simulink model "afe_rst_inv_psm_distributed_control_two_delays"  (R2026a)
settings: Solver=ode1be  StopTime=simlength  FixedStep=tc  MaxStep=Tc
values from neighbouring files (symbols this model uses):
  Amplitude_U = 1.16    [grid_fault_generator.m]
  Amplitude_V = Amplitude_U    (= 1.16)    [grid_fault_generator.m]
  Amplitude_W = Amplitude_U    (= 1.16)    [grid_fault_generator.m]
  end_time_LVRT = start_time_LVRT + error_length    [grid_fault_generator.m]
  Igrid_phase_normalization_factor = 270*sqrt(2)    [grid_emulator.m]
  omega_grid_emulator_nom = w_grid    (= 314.159265359)    [grid_emulator.m]
  omega_grid_nom = w_grid    (= 314.159265359)    [grid_emulator.m]
  t_ramp = 20e-3    (= 0.02)    [grid_fault_generator.m]
  ugrid_factor = 1    [grid_emulator.m]
  V_phase_normalization_factor = Vgrid_phase_normalization_factor    [grid_emulator.m]
  Vdc_bez = 1070    [grid_emulator.m]
  Vemu_ref_norm = Vemu_ref * sqrt(2) / V_phase_normalization_factor    [grid_emulator.m]
  vn_eta_pu = 0    [grid_emulator.m]
  vn_xi_pu = 0    [grid_emulator.m]
  vp_xi_pu = 1    [grid_emulator.m]
undefined symbols (not defined in the file or in its folder): Adrso, Aresd, Bresd, CFi, CFu, Cresd, Crso, CTRPIFF_CLIP_RELEASE, dead_time_INV, emf_fb_p, emf_fb_p_ccaller_1, emf_fb_p_ccaller_2, emf_p, emf_p_ccaller_1, emf_p_ccaller_2, fPWM_INV, g0_161Hz, g0_500Hz, g1_161Hz, g1_500Hz, i_grid_neg_eta_lim, i_grid_neg_eta_red_lim, i_grid_neg_xi_lim, i_grid_neg_xi_red_lim, i_grid_pos_eta_lim, i_grid_pos_eta_red_lim, ibez, id_lim, ieta_neg_ref_lim, ieta_pos_ref_lim, iq_lim, ixi_pos_ref_lim, Jm_norm, k_frt_ref, kg, ki_afe, ki_i, ki_id, ki_iq, ki_rc_neg_grid, ki_rc_pos_grid, ki_vs, ki_w, kp_afe, kp_i, kp_id, kp_iq, kp_rc_neg_grid, kp_rc_pos_grid, kp_vs, kp_w, kw, l1, l2, Lalpha_norm, Ld_norm, Ldrso, Lq_norm, Ls_norm, luenberger_l1 ... (+30)
libraries: fl_lib x146, nesl_utility x62, simulink x8, cstblocks_lti x7, sl_discontinuities x3, single_phase_transformer_lib x3, flexshaft_lib x1, permanent_magnet_synchronous_machine x1
(part 3 of 14)

== system afe_rst_inv_psm_distributed_control_two_delays/AFE-Modular/afe_leg_a/solid_state_inverter ==
  Simulink-PS Converter : nesl_utility/Simulink-PS Converter  PhysicalDomain=network_engine_domain  SubClassName=ps_input  LeftPortType=input  RightPortType=output  PseudoPeriodic=off  Frequencies=[]  NoiseDistribution=none  NoiseParameters=[]  Unit=1  AffineConversion=off  FilteringAndDerivatives=provide  SimscapeFilterOrder=1  InputFilterTimeConstant=0.001  UdotUserProvided=0
  Simulink-PS Converter1 : nesl_utility/Simulink-PS Converter  PhysicalDomain=network_engine_domain  SubClassName=ps_input  LeftPortType=input  RightPortType=output  PseudoPeriodic=off  Frequencies=[]  NoiseDistribution=none  NoiseParameters=[]  Unit=1  AffineConversion=off  FilteringAndDerivatives=provide  SimscapeFilterOrder=1  InputFilterTimeConstant=0.001  UdotUserProvided=0
  switch_1 : Subsystem
      settings: PortSchema="{\"entries\":[{\"content\":{\"sides\":[{\"content\":{\"connectorIds\":[\"LConn1\"]},\"type\":\"ConnectorPlacement.EquallySpacedRectSide\",\"uuid\":\"9277da8d-d460-43e6-8478-dd662f15d226\"},{\"content\":{\"connectorIds\":[],\"side\":\"RIGHT\"},\"type\":\"ConnectorPlacement.EquallySpacedRectSide\",\"uuid\":\"a7ece396-f1d9-4f4f-a05b-db1fc65d6e1d\"},{\"content\":{\"connectorIds\":[\"LConn2\"],\"side\":\"TOP\"},\"type\":\"ConnectorPlacement.EquallySpacedRectSide\",\"uuid\":\"fdd70777-e9cf-4317-afb6-cae87f75d5b0\"},{\"content\":{\"connectorIds\":[\"RConn1\"],\"side\":\"BOTTOM\"},\"type\":\"ConnectorPlacement.EquallySpacedRectSide\",\"uuid\":\"2353ed68-b1a1-4775-9ca9-31e268d5443b\"}]},\"type\":\"ConnectorPlacement.EquallySpacedConnector\",\"uuid\":\"d5479f4c-4e65-4791-adcb-73df11f88590\"}],\"packageUris\":[\"http://schema.mathworks.com/mf0/Connector/R2020b\"],\"version\":\"1.0\"}"
  switch_2 : Subsystem
      settings: PortSchema="{\"entries\":[{\"content\":{\"sides\":[{\"content\":{\"connectorIds\":[\"LConn1\"]},\"type\":\"ConnectorPlacement.EquallySpacedRectSide\",\"uuid\":\"9277da8d-d460-43e6-8478-dd662f15d226\"},{\"content\":{\"connectorIds\":[],\"side\":\"RIGHT\"},\"type\":\"ConnectorPlacement.EquallySpacedRectSide\",\"uuid\":\"a7ece396-f1d9-4f4f-a05b-db1fc65d6e1d\"},{\"content\":{\"connectorIds\":[\"LConn2\"],\"side\":\"TOP\"},\"type\":\"ConnectorPlacement.EquallySpacedRectSide\",\"uuid\":\"fdd70777-e9cf-4317-afb6-cae87f75d5b0\"},{\"content\":{\"connectorIds\":[\"RConn1\"],\"side\":\"BOTTOM\"},\"type\":\"ConnectorPlacement.EquallySpacedRectSide\",\"uuid\":\"2353ed68-b1a1-4775-9ca9-31e268d5443b\"}]},\"type\":\"ConnectorPlacement.EquallySpacedConnector\",\"uuid\":\"d5479f4c-4e65-4791-adcb-73df11f88590\"}],\"packageUris\":[\"http://schema.mathworks.com/mf0/Connector/R2020b\"],\"version\":\"1.0\"}"
  Udc(+) : PMIOPort  Side=Left
  us_a : PMIOPort  Port=2  Side=Right
  Udc(-) : PMIOPort  Port=3  Side=Left
  wires:
  [afe_mu_bottom] -> Simulink-PS Converter1/1
  [afe_mu_top] -> Simulink-PS Converter/1
  connections:
  Udc(-)/RConn1 -- switch_2/RConn1
  switch_1/RConn1 -- switch_2/LConn2 -- us_a/RConn1
  Simulink-PS Converter/RConn1 -- switch_1/LConn1
  switch_2/LConn1 -- Simulink-PS Converter1/RConn1
  Udc(+)/RConn1 -- switch_1/LConn2

== system afe_rst_inv_psm_distributed_control_two_delays/AFE-Modular/afe_leg_b/dclink_measure ==
  Controlled Voltage Source : fl_lib/Electrical/Electrical Sources/Controlled Voltage Source
  Current Sensor1 : fl_lib/Electrical/Electrical Sensors/Current Sensor
  Electrical Reference : fl_lib/Electrical/Electrical Elements/Electrical Reference
  Gain : Gain  Gain=107.5e3
  Gain1 : Gain  Gain=1/Vdc_bez
  Quantizer : Quantizer  QuantizationInterval=VoltageQuantization
  Resistor : fl_lib/Electrical/Electrical Elements/Resistor  R=107.5 kOhm  i_specify=off  i_priority=None  i=0 A  i_nominal_specify=off  i_nominal_value=1  i_nominal_unit=A  v_specify=off  v_priority=None  v=0 V  v_nominal_specify=off  v_nominal_value=1  v_nominal_unit=V
  Saturation : Saturate  UpperLimit=inf  LowerLimit=1
  im_udc : nesl_utility/PS-Simulink Converter  PhysicalDomain=network_engine_domain  SubClassName=ps_output  LeftPortType=input  RightPortType=output  PseudoPeriodic=off  Frequencies=[]  VectorFormat=1-D array  Unit=A  AffineConversion=on
  udc : PMIOPort  Side=Left
  tag scope: udc_pu_phase_b=global
  wires:
  Gain1/1 -> [udc_pu_phase_b]
  im_udc/1 -> Gain/1
  Saturation/1 -> Quantizer/1
  Quantizer/1 -> Gain1/1
  Gain/1 -> Saturation/1
  connections:
  Controlled Voltage Source/LConn1 -- Resistor/LConn1
  Resistor/RConn1 -- Current Sensor1/LConn1
  Controlled Voltage Source/RConn2 -- Electrical Reference/LConn1 -- Current Sensor1/RConn2
  Current Sensor1/RConn1 -- im_udc/LConn1
  udc/RConn1 -- Controlled Voltage Source/RConn1

== system afe_rst_inv_psm_distributed_control_two_delays/AFE-Modular/afe_leg_b/driver_board_b ==
  current_ctrl : Subsystem
  dq_pll : Subsystem
  igb_dbb_estimator : Subsystem
  voltage-current-acquisition : Subsystem
  us_alphabeta_ctrl : Outport
  wires:
  current_ctrl/1(us_alphabeta_ctrl) -> us_alphabeta_ctrl/1
  [ixi_ref_dba_fb_dbb] -> current_ctrl/1(i_xi_ref)

== system afe_rst_inv_psm_distributed_control_two_delays/AFE-Modular/afe_leg_b/modulator ==
  us_alphabeta_ctrl : Inport
  Bus Selector : BusSelector  OutputSignals=pwm_v_top,pwm_v_bottom
  Constant1 : Constant
  sv_pwm : Subsystem
  tag scope: afe_mv_bottom=global, afe_mv_top=global
  wires:
  sv_pwm/1(firing_gates) -> Bus Selector/1
  Constant1/1 -> sv_pwm/2(enable)
  Bus Selector/1 -> [afe_mv_top]  "<pwm_v_top>"
  us_alphabeta_ctrl/1 -> sv_pwm/1(ab)
  Bus Selector/2 -> [afe_mv_bottom]  "<pwm_v_bottom>"

== system afe_rst_inv_psm_distributed_control_two_delays/AFE-Modular/afe_leg_b/solid_state_inverter ==
  Simulink-PS Converter : nesl_utility/Simulink-PS Converter  PhysicalDomain=network_engine_domain  SubClassName=ps_input  LeftPortType=input  RightPortType=output  PseudoPeriodic=off  Frequencies=[]  NoiseDistribution=none  NoiseParameters=[]  Unit=1  AffineConversion=off  FilteringAndDerivatives=provide  SimscapeFilterOrder=1  InputFilterTimeConstant=0.001  UdotUserProvided=0
  Simulink-PS Converter1 : nesl_utility/Simulink-PS Converter  PhysicalDomain=network_engine_domain  SubClassName=ps_input  LeftPortType=input  RightPortType=output  PseudoPeriodic=off  Frequencies=[]  NoiseDistribution=none  NoiseParameters=[]  Unit=1  AffineConversion=off  FilteringAndDerivatives=provide  SimscapeFilterOrder=1  InputFilterTimeConstant=0.001  UdotUserProvided=0
  switch_1 : Subsystem
      settings: PortSchema="{\"entries\":[{\"content\":{\"sides\":[{\"content\":{\"connectorIds\":[\"LConn1\"]},\"type\":\"ConnectorPlacement.EquallySpacedRectSide\",\"uuid\":\"9277da8d-d460-43e6-8478-dd662f15d226\"},{\"content\":{\"connectorIds\":[],\"side\":\"RIGHT\"},\"type\":\"ConnectorPlacement.EquallySpacedRectSide\",\"uuid\":\"a7ece396-f1d9-4f4f-a05b-db1fc65d6e1d\"},{\"content\":{\"connectorIds\":[\"LConn2\"],\"side\":\"TOP\"},\"type\":\"ConnectorPlacement.EquallySpacedRectSide\",\"uuid\":\"fdd70777-e9cf-4317-afb6-cae87f75d5b0\"},{\"content\":{\"connectorIds\":[\"RConn1\"],\"side\":\"BOTTOM\"},\"type\":\"ConnectorPlacement.EquallySpacedRectSide\",\"uuid\":\"2353ed68-b1a1-4775-9ca9-31e268d5443b\"}]},\"type\":\"ConnectorPlacement.EquallySpacedConnector\",\"uuid\":\"d5479f4c-4e65-4791-adcb-73df11f88590\"}],\"packageUris\":[\"http://schema.mathworks.com/mf0/Connector/R2020b\"],\"version\":\"1.0\"}"
  switch_2 : Subsystem
      settings: PortSchema="{\"entries\":[{\"content\":{\"sides\":[{\"content\":{\"connectorIds\":[\"LConn1\"]},\"type\":\"ConnectorPlacement.EquallySpacedRectSide\",\"uuid\":\"9277da8d-d460-43e6-8478-dd662f15d226\"},{\"content\":{\"connectorIds\":[],\"side\":\"RIGHT\"},\"type\":\"ConnectorPlacement.EquallySpacedRectSide\",\"uuid\":\"a7ece396-f1d9-4f4f-a05b-db1fc65d6e1d\"},{\"content\":{\"connectorIds\":[\"LConn2\"],\"side\":\"TOP\"},\"type\":\"ConnectorPlacement.EquallySpacedRectSide\",\"uuid\":\"fdd70777-e9cf-4317-afb6-cae87f75d5b0\"},{\"content\":{\"connectorIds\":[\"RConn1\"],\"side\":\"BOTTOM\"},\"type\":\"ConnectorPlacement.EquallySpacedRectSide\",\"uuid\":\"2353ed68-b1a1-4775-9ca9-31e268d5443b\"}]},\"type\":\"ConnectorPlacement.EquallySpacedConnector\",\"uuid\":\"d5479f4c-4e65-4791-adcb-73df11f88590\"}],\"packageUris\":[\"http://schema.mathworks.com/mf0/Connector/R2020b\"],\"version\":\"1.0\"}"
  Udc(+) : PMIOPort  Side=Left
  us_b : PMIOPort  Port=2  Side=Right
  Udc(-) : PMIOPort  Port=3  Side=Left
  wires:
  [afe_mv_top] -> Simulink-PS Converter/1
  [afe_mv_bottom] -> Simulink-PS Converter1/1
  connections:
  Udc(+)/RConn1 -- switch_1/LConn2
  switch_2/LConn1 -- Simulink-PS Converter1/RConn1
  Simulink-PS Converter/RConn1 -- switch_1/LConn1
  switch_2/LConn2 -- us_b/RConn1 -- switch_1/RConn1
  Udc(-)/RConn1 -- switch_2/RConn1

== system afe_rst_inv_psm_distributed_control_two_delays/AFE-Modular/afe_leg_c/dclink_measure ==
  Controlled Voltage Source : fl_lib/Electrical/Electrical Sources/Controlled Voltage Source
  Current Sensor1 : fl_lib/Electrical/Electrical Sensors/Current Sensor
  Electrical Reference : fl_lib/Electrical/Electrical Elements/Electrical Reference
  Gain : Gain  Gain=107.5e3
  Gain1 : Gain  Gain=1/Vdc_bez
  Quantizer : Quantizer  QuantizationInterval=VoltageQuantization
  Resistor : fl_lib/Electrical/Electrical Elements/Resistor  R=107.5 kOhm  i_specify=off  i_priority=None  i=0 A  i_nominal_specify=off  i_nominal_value=1  i_nominal_unit=A  v_specify=off  v_priority=None  v=0 V  v_nominal_specify=off  v_nominal_value=1  v_nominal_unit=V
  Saturation : Saturate  UpperLimit=inf  LowerLimit=1
  im_udc : nesl_utility/PS-Simulink Converter  PhysicalDomain=network_engine_domain  SubClassName=ps_output  LeftPortType=input  RightPortType=output  PseudoPeriodic=off  Frequencies=[]  VectorFormat=1-D array  Unit=A  AffineConversion=on
  udc : PMIOPort  Side=Left
  tag scope: vdc_pu=global
  wires:
  Gain/1 -> Saturation/1
  Quantizer/1 -> Gain1/1
  Saturation/1 -> Quantizer/1
  im_udc/1 -> Gain/1
  Gain1/1 -> [vdc_pu]
  connections:
  udc/RConn1 -- Controlled Voltage Source/RConn1
  Current Sensor1/RConn1 -- im_udc/LConn1
  Current Sensor1/RConn2 -- Electrical Reference/LConn1 -- Controlled Voltage Source/RConn2
  Resistor/RConn1 -- Current Sensor1/LConn1
  Controlled Voltage Source/LConn1 -- Resistor/LConn1

== system afe_rst_inv_psm_distributed_control_two_delays/AFE-Modular/afe_leg_c/driver_board_c ==
  current_ctrl : Subsystem
  dq_pll : Subsystem
  igc_dbc_estimator : Subsystem
  voltage-current-acquisition : Subsystem
  us_alphabeta_ctrl : Outport
  wires:
  current_ctrl/1(us_alphabeta_ctrl) -> us_alphabeta_ctrl/1
  [ixi_ref_dba_fb_dbc] -> current_ctrl/1(i_xi_ref)

== system afe_rst_inv_psm_distributed_control_two_delays/AFE-Modular/afe_leg_c/modulator ==
  u_alphabeta_ctrl : Inport
  Bus Selector : BusSelector  OutputSignals=pwm_w_top,pwm_w_bottom
  Constant1 : Constant
  sv_pwm : Subsystem
  tag scope: afe_mw_bottom=global, afe_mw_top=global
  wires:
  Bus Selector/2 -> [afe_mw_bottom]  "<pwm_w_bottom>"
  u_alphabeta_ctrl/1 -> sv_pwm/1(u_alphabeta_ctrl)
  Bus Selector/1 -> [afe_mw_top]  "<pwm_w_top>"
  Constant1/1 -> sv_pwm/2(enable)
  sv_pwm/1(firing_gates) -> Bus Selector/1

== system afe_rst_inv_psm_distributed_control_two_delays/AFE-Modular/afe_leg_c/solid_state_inverter ==
  Simulink-PS Converter : nesl_utility/Simulink-PS Converter  PhysicalDomain=network_engine_domain  SubClassName=ps_input  LeftPortType=input  RightPortType=output  PseudoPeriodic=off  Frequencies=[]  NoiseDistribution=none  NoiseParameters=[]  Unit=1  AffineConversion=off  FilteringAndDerivatives=provide  SimscapeFilterOrder=1  InputFilterTimeConstant=0.001  UdotUserProvided=0
  Simulink-PS Converter1 : nesl_utility/Simulink-PS Converter  PhysicalDomain=network_engine_domain  SubClassName=ps_input  LeftPortType=input  RightPortType=output  PseudoPeriodic=off  Frequencies=[]  NoiseDistribution=none  NoiseParameters=[]  Unit=1  AffineConversion=off  FilteringAndDerivatives=provide  SimscapeFilterOrder=1  InputFilterTimeConstant=0.001  UdotUserProvided=0
  switch_1 : Subsystem
      settings: PortSchema="{\"entries\":[{\"content\":{\"sides\":[{\"content\":{\"connectorIds\":[\"LConn1\"]},\"type\":\"ConnectorPlacement.EquallySpacedRectSide\",\"uuid\":\"9277da8d-d460-43e6-8478-dd662f15d226\"},{\"content\":{\"connectorIds\":[],\"side\":\"RIGHT\"},\"type\":\"ConnectorPlacement.EquallySpacedRectSide\",\"uuid\":\"a7ece396-f1d9-4f4f-a05b-db1fc65d6e1d\"},{\"content\":{\"connectorIds\":[\"LConn2\"],\"side\":\"TOP\"},\"type\":\"ConnectorPlacement.EquallySpacedRectSide\",\"uuid\":\"fdd70777-e9cf-4317-afb6-cae87f75d5b0\"},{\"content\":{\"connectorIds\":[\"RConn1\"],\"side\":\"BOTTOM\"},\"type\":\"ConnectorPlacement.EquallySpacedRectSide\",\"uuid\":\"2353ed68-b1a1-4775-9ca9-31e268d5443b\"}]},\"type\":\"ConnectorPlacement.EquallySpacedConnector\",\"uuid\":\"d5479f4c-4e65-4791-adcb-73df11f88590\"}],\"packageUris\":[\"http://schema.mathworks.com/mf0/Connector/R2020b\"],\"version\":\"1.0\"}"
  switch_2 : Subsystem
      settings: PortSchema="{\"entries\":[{\"content\":{\"sides\":[{\"content\":{\"connectorIds\":[\"LConn1\"]},\"type\":\"ConnectorPlacement.EquallySpacedRectSide\",\"uuid\":\"9277da8d-d460-43e6-8478-dd662f15d226\"},{\"content\":{\"connectorIds\":[],\"side\":\"RIGHT\"},\"type\":\"ConnectorPlacement.EquallySpacedRectSide\",\"uuid\":\"a7ece396-f1d9-4f4f-a05b-db1fc65d6e1d\"},{\"content\":{\"connectorIds\":[\"LConn2\"],\"side\":\"TOP\"},\"type\":\"ConnectorPlacement.EquallySpacedRectSide\",\"uuid\":\"fdd70777-e9cf-4317-afb6-cae87f75d5b0\"},{\"content\":{\"connectorIds\":[\"RConn1\"],\"side\":\"BOTTOM\"},\"type\":\"ConnectorPlacement.EquallySpacedRectSide\",\"uuid\":\"2353ed68-b1a1-4775-9ca9-31e268d5443b\"}]},\"type\":\"ConnectorPlacement.EquallySpacedConnector\",\"uuid\":\"d5479f4c-4e65-4791-adcb-73df11f88590\"}],\"packageUris\":[\"http://schema.mathworks.com/mf0/Connector/R2020b\"],\"version\":\"1.0\"}"
  Udc(+) : PMIOPort  Side=Left
  us_b : PMIOPort  Port=2  Side=Right
  Udc(-) : PMIOPort  Port=3  Side=Left
  wires:
  [afe_mw_bottom] -> Simulink-PS Converter1/1
  [afe_mw_top] -> Simulink-PS Converter/1
  connections:
  Udc(-)/RConn1 -- switch_2/RConn1
  switch_1/RConn1 -- us_b/RConn1 -- switch_2/LConn2
  Simulink-PS Converter/RConn1 -- switch_1/LConn1
  switch_2/LConn1 -- Simulink-PS Converter1/RConn1
  Udc(+)/RConn1 -- switch_1/LConn2

== system afe_rst_inv_psm_distributed_control_two_delays/FRT-VDE4110/FRT-Detection/dvxi_n//dt ==
  x : Inport
  Gain : Gain  Gain=l2
  Gain1 : Gain  Gain=l1
  Gain5 : Gain  Gain=ts_afe
  Sum : Sum  Inputs=-+|
  Sum1 : Sum  Inputs=|++
  Sum2 : Sum  Inputs=|++
  Sum8 : Sum  Inputs=++|
  Unit Delay1 : UnitDelay  SampleTime=ts_afe
  Unit Delay2 : UnitDelay  SampleTime=ts_afe
  xdot_hat : Outport  VectorParamsAs1DForOutWhenUnconnected=off
  wires:
  Unit Delay2/1 -> Gain5/1, Sum1/2, xdot_hat/1
  Sum8/1 -> Unit Delay1/1
  Sum/1 -> Gain/1, Gain1/1
  Unit Delay1/1 -> Sum/1, Sum2/2  "x_hat"
  Sum2/1 -> Sum8/2
  Gain/1 -> Sum1/1
  Sum1/1 -> Unit Delay2/1
  Gain5/1 -> Sum8/1
  x/1 -> Sum/2  "x"
  Gain1/1 -> Sum2/1

== system afe_rst_inv_psm_distributed_control_two_delays/FRT-VDE4110/FRT-Detection/dvxi_p//dt ==
  x : Inport
  Gain : Gain  Gain=l2
  Gain1 : Gain  Gain=l1
  Gain5 : Gain  Gain=ts_afe
  Sum : Sum  Inputs=-+|
  Sum1 : Sum  Inputs=|++
  Sum2 : Sum  Inputs=|++
  Sum8 : Sum  Inputs=++|
  Unit Delay1 : UnitDelay  SampleTime=ts_afe
  Unit Delay2 : UnitDelay  SampleTime=ts_afe
  xdot_hat : Outport  VectorParamsAs1DForOutWhenUnconnected=off
  wires:
  Gain1/1 -> Sum2/1
  x/1 -> Sum/2  "x"
  Gain5/1 -> Sum8/1
  Sum1/1 -> Unit Delay2/1
  Gain/1 -> Sum1/1
  Sum2/1 -> Sum8/2
  Unit Delay1/1 -> Sum2/2, Sum/1  "x_hat"
  Sum/1 -> Gain1/1, Gain/1
  Sum8/1 -> Unit Delay1/1
  Unit Delay2/1 -> xdot_hat/1, Sum1/2, Gain5/1

== system afe_rst_inv_psm_distributed_control_two_delays/FRT-VDE4110/FRT-PosNegReactiveCurrentReferences/avg_flt_500ms ==
  note: Bei fehler: Alter Grid-Wert wird festgehalten!!
  In1 : Inport
  Constant : Constant  Value=2*pi/500e-3
  Constant1 : Constant  Value=ts_afe
  Constant2 : Constant
  Sum : Sum  Inputs=|-+
  avg_flt_1 : MATLAB Function  TreatAsAtomicUnit=on  SystemSampleTime=ts_afe
  Out1 : Outport  VectorParamsAs1DForOutWhenUnconnected=off
  wires:
  avg_flt_1/1(y1) -> Out1/1  "output"
  Constant1/1 -> avg_flt_1/3(Tc)
  Constant/1 -> avg_flt_1/2(w)
  In1/1 -> avg_flt_1/1(x)  "input"
  Constant2/1 -> Sum/2
  [frt_active] -> Sum/1
  Sum/1 -> avg_flt_1/4(enable)

== system afe_rst_inv_psm_distributed_control_two_delays/FRT-VDE4110/FRT-PosNegReactiveCurrentReferences/avg_flt_500ms1 ==
  note: Bei fehler: Alter Grid-Wert wird festgehalten!!
  In1 : Inport
  Constant : Constant  Value=2*pi/500e-3
  Constant1 : Constant  Value=ts_afe
  avg_flt_1 : MATLAB Function  TreatAsAtomicUnit=on  SystemSampleTime=ts_afe
  Out1 : Outport  VectorParamsAs1DForOutWhenUnconnected=off
  wires:
  avg_flt_1/1(y1) -> Out1/1  "output"
  Constant1/1 -> avg_flt_1/3(Tc)
  Constant/1 -> avg_flt_1/2(w)
  In1/1 -> avg_flt_1/1(x)  "input"
  [frt_active] -> avg_flt_1/4(enable)

== system afe_rst_inv_psm_distributed_control_two_delays/FRT-VDE4110/FRT-PosNegReactiveCurrentReferences/avg_flt_500ms2 ==
  note: Bei fehler: Alter Grid-Wert wird festgehalten!!
  In1 : Inport
  Constant : Constant  Value=2*pi/500e-3
  Constant1 : Constant  Value=ts_afe
  Constant2 : Constant
  Sum : Sum  Inputs=|-+
  avg_flt_1 : MATLAB Function  TreatAsAtomicUnit=on  SystemSampleTime=ts_afe
  Out1 : Outport  VectorParamsAs1DForOutWhenUnconnected=off
  wires:
  avg_flt_1/1(y1) -> Out1/1  "output"
  Constant1/1 -> avg_flt_1/3(Tc)
  Constant/1 -> avg_flt_1/2(w)
  In1/1 -> avg_flt_1/1(x)  "input"
  Constant2/1 -> Sum/2
  [frt_active] -> Sum/1
  Sum/1 -> avg_flt_1/4(enable)

== system afe_rst_inv_psm_distributed_control_two_delays/FRT-VDE4110/FRT-PosNegReactiveCurrentReferences/avg_flt_500ms3 ==
  note: Bei fehler: Alter Grid-Wert wird festgehalten!!
  In1 : Inport
  Constant : Constant  Value=2*pi/500e-3
  Constant1 : Constant  Value=ts_afe
  Constant2 : Constant
  Sum : Sum  Inputs=|-+
  avg_flt_1 : MATLAB Function  TreatAsAtomicUnit=on  SystemSampleTime=ts_afe
  Out1 : Outport  VectorParamsAs1DForOutWhenUnconnected=off
  wires:
  avg_flt_1/1(y1) -> Out1/1  "output"
  Constant1/1 -> avg_flt_1/3(Tc)
  Constant/1 -> avg_flt_1/2(w)
  In1/1 -> avg_flt_1/1(x)  "input"
  [frt_active] -> Sum/1
  Constant2/1 -> Sum/2
  Sum/1 -> avg_flt_1/4(enable)

== system afe_rst_inv_psm_distributed_control_two_delays/FRT-VDE4110/FRT-PosNegReactiveCurrentReferences/u_161Hz_flt1 ==
  input : Inport
  Gain3 : Gain  Gain=g1_161Hz
  Gain6 : Gain  Gain=g0_161Hz
  Sum : Sum  Inputs=|++
  Unit Delay1 : UnitDelay  SampleTime=ts_afe
  output : Outport  VectorParamsAs1DForOutWhenUnconnected=off
  wires:
  Gain6/1 -> Sum/1
  input/1 -> Gain6/1
  Unit Delay1/1 -> Gain3/1
  Gain3/1 -> Sum/2
  Sum/1 -> Unit Delay1/1, output/1

== system afe_rst_inv_psm_distributed_control_two_delays/FRT-VDE4110/FRT-PosNegReactiveCurrentReferences/u_161Hz_flt2 ==
  input : Inport
  Gain3 : Gain  Gain=g1_161Hz
  Gain6 : Gain  Gain=g0_161Hz
  Sum : Sum  Inputs=|++
  Unit Delay1 : UnitDelay  SampleTime=ts_afe
  output : Outport  VectorParamsAs1DForOutWhenUnconnected=off
  wires:
  Sum/1 -> output/1, Unit Delay1/1
  Gain3/1 -> Sum/2
  Unit Delay1/1 -> Gain3/1
  input/1 -> Gain6/1
  Gain6/1 -> Sum/1

== system afe_rst_inv_psm_distributed_control_two_delays/FRT-VDE4110/FRT-PosNegReactiveCurrentReferences/u_161Hz_flt3 ==
  input : Inport
  Gain3 : Gain  Gain=g1_161Hz
  Gain6 : Gain  Gain=g0_161Hz
  Sum : Sum  Inputs=|++
  Unit Delay1 : UnitDelay  SampleTime=ts_afe
  output : Outport  VectorParamsAs1DForOutWhenUnconnected=off
  wires:
  Gain6/1 -> Sum/1
  input/1 -> Gain6/1
  Unit Delay1/1 -> Gain3/1
  Gain3/1 -> Sum/2
  Sum/1 -> Unit Delay1/1, output/1

== system afe_rst_inv_psm_distributed_control_two_delays/INV-Modular/inv_leg_u/dclink_measure ==
  Controlled Voltage Source : fl_lib/Electrical/Electrical Sources/Controlled Voltage Source
  Current Sensor1 : fl_lib/Electrical/Electrical Sensors/Current Sensor
  Electrical Reference : fl_lib/Electrical/Electrical Elements/Electrical Reference
  Gain : Gain  Gain=107.5e3
  Gain1 : Gain  Gain=1/Vdc_bez
  Quantizer : Quantizer  QuantizationInterval=VoltageQuantization
  Resistor : fl_lib/Electrical/Electrical Elements/Resistor  R=107.5 kOhm  i_specify=off  i_priority=None  i=0 A  i_nominal_specify=off  i_nominal_value=1  i_nominal_unit=A  v_specify=off  v_priority=None  v=0 V  v_nominal_specify=off  v_nominal_value=1  v_nominal_unit=V
  Saturation : Saturate  UpperLimit=inf  LowerLimit=1
  im_udc : nesl_utility/PS-Simulink Converter  PhysicalDomain=network_engine_domain  SubClassName=ps_output  LeftPortType=input  RightPortType=output  PseudoPeriodic=off  Frequencies=[]  VectorFormat=1-D array  Unit=A  AffineConversion=on
  udc : PMIOPort  Side=Left
  tag scope: udc_dbu=global, udc_pu_dbu=global
  wires:
  Gain/1 -> [udc_dbu], Saturation/1
  Quantizer/1 -> Gain1/1
  Saturation/1 -> Quantizer/1
  im_udc/1 -> Gain/1
  Gain1/1 -> [udc_pu_dbu]
  connections:
  udc/RConn1 -- Controlled Voltage Source/RConn1
  Current Sensor1/RConn1 -- im_udc/LConn1
  Current Sensor1/RConn2 -- Electrical Reference/LConn1 -- Controlled Voltage Source/RConn2
  Resistor/RConn1 -- Current Sensor1/LConn1
  Controlled Voltage Source/LConn1 -- Resistor/LConn1

== system afe_rst_inv_psm_distributed_control_two_delays/INV-Modular/inv_leg_u/driver_board_u ==
  Gain : Gain  Gain=1/omega_bez
  Rate Limiter : RateLimiter  SampleTimeMode=inherited
  Step : Step  Time=0.1  SampleTime=0
  Variant Source : VariantSource  VariantControls={motor_torque_mode == 0, motor_torque_mode == 1}
  double_integrator_observer : Subsystem
  motor_vector_control : Subsystem
  psm_speed_ctrl : Subsystem
  torque_curve : Subsystem
  torque_curve_pu : Scope  NumInputPorts=3
      settings: SampleTime=tc  ActiveDisplayYMinimum=-1.1044  ActiveDisplayYMaximum=0.12271
  voltage-current-acquisition : Subsystem
  us_alphabeta_ctrl : Outport
  tag scope: motor_phase_mb_fb_dbu_luenberger=global, motor_torque_ref_dbu=global
  wires:
  Step/1 -> Rate Limiter/1
  double_integrator_observer/1(omega_pu_hat) -> psm_speed_ctrl/1(motor_omega)
  motor_vector_control/1(us_alphabeta_ctrl) -> us_alphabeta_ctrl/1
  Rate Limiter/1 -> psm_speed_ctrl/2(motor_omega_ref)
  [motor_phase_mb_fb_dbu] -> double_integrator_observer/1(theta)
  double_integrator_observer/2(theta_hat) -> [motor_phase_mb_fb_dbu_luenberger]  "theta_hat"
  [motor_omega_hat_pu_dbu] -> torque_curve_pu/2, torque_curve/1(rotor speed)  "motor_speed_pu_hat"
  Variant Source/1 -> [motor_torque_ref_dbu], motor_vector_control/1(motor_torque_ref)
  psm_speed_ctrl/1(motor_torque_ref) -> Variant Source/1  "motor_torque_pu_ref"
  torque_curve/1(torque_ref) -> Variant Source/2, torque_curve_pu/1  "motor_torque_pu_ref"
  [omega_elec_pmsm] -> Gain/1
  Gain/1 -> torque_curve_pu/3  "motor_speed_pu"

== system afe_rst_inv_psm_distributed_control_two_delays/INV-Modular/inv_leg_u/modulator ==
  us_alphabeta_ctrl : Inport
  Bus Selector : BusSelector  OutputSignals=pwm_u_top,pwm_u_bottom
  Constant1 : Constant
  sv_pwm : Subsystem
  tag scope: inv_mu_bottom=global, inv_mu_top=global
  wires:
  sv_pwm/1(firing_gates) -> Bus Selector/1
  Constant1/1 -> sv_pwm/2(enable)
  Bus Selector/1 -> [inv_mu_top]  "<pwm_u_top>"
  us_alphabeta_ctrl/1 -> sv_pwm/1(ab)
  Bus Selector/2 -> [inv_mu_bottom]  "<pwm_u_bottom>"

== system afe_rst_inv_psm_distributed_control_two_delays/INV-Modular/inv_leg_u/solid_state_inverter ==
  Simulink-PS Converter : nesl_utility/Simulink-PS Converter  PhysicalDomain=network_engine_domain  SubClassName=ps_input  LeftPortType=input  RightPortType=output  PseudoPeriodic=off  Frequencies=[]  NoiseDistribution=none  NoiseParameters=[]  Unit=1  AffineConversion=off  FilteringAndDerivatives=provide  SimscapeFilterOrder=1  InputFilterTimeConstant=0.001  UdotUserProvided=0
  Simulink-PS Converter1 : nesl_utility/Simulink-PS Converter  PhysicalDomain=network_engine_domain  SubClassName=ps_input  LeftPortType=input  RightPortType=output  PseudoPeriodic=off  Frequencies=[]  NoiseDistribution=none  NoiseParameters=[]  Unit=1  AffineConversion=off  FilteringAndDerivatives=provide  SimscapeFilterOrder=1  InputFilterTimeConstant=0.001  UdotUserProvided=0
  switch_1 : Subsystem
      settings: PortSchema="{\"entries\":[{\"content\":{\"sides\":[{\"content\":{\"connectorIds\":[\"LConn1\"]},\"type\":\"ConnectorPlacement.EquallySpacedRectSide\",\"uuid\":\"9277da8d-d460-43e6-8478-dd662f15d226\"},{\"content\":{\"connectorIds\":[],\"side\":\"RIGHT\"},\"type\":\"ConnectorPlacement.EquallySpacedRectSide\",\"uuid\":\"a7ece396-f1d9-4f4f-a05b-db1fc65d6e1d\"},{\"content\":{\"connectorIds\":[\"LConn2\"],\"side\":\"TOP\"},\"type\":\"ConnectorPlacement.EquallySpacedRectSide\",\"uuid\":\"fdd70777-e9cf-4317-afb6-cae87f75d5b0\"},{\"content\":{\"connectorIds\":[\"RConn1\"],\"side\":\"BOTTOM\"},\"type\":\"ConnectorPlacement.EquallySpacedRectSide\",\"uuid\":\"2353ed68-b1a1-4775-9ca9-31e268d5443b\"}]},\"type\":\"ConnectorPlacement.EquallySpacedConnector\",\"uuid\":\"d5479f4c-4e65-4791-adcb-73df11f88590\"}],\"packageUris\":[\"http://schema.mathworks.com/mf0/Connector/R2020b\"],\"version\":\"1.0\"}"
  switch_2 : Subsystem
      settings: PortSchema="{\"entries\":[{\"content\":{\"sides\":[{\"content\":{\"connectorIds\":[\"LConn1\"]},\"type\":\"ConnectorPlacement.EquallySpacedRectSide\",\"uuid\":\"9277da8d-d460-43e6-8478-dd662f15d226\"},{\"content\":{\"connectorIds\":[],\"side\":\"RIGHT\"},\"type\":\"ConnectorPlacement.EquallySpacedRectSide\",\"uuid\":\"a7ece396-f1d9-4f4f-a05b-db1fc65d6e1d\"},{\"content\":{\"connectorIds\":[\"LConn2\"],\"side\":\"TOP\"},\"type\":\"ConnectorPlacement.EquallySpacedRectSide\",\"uuid\":\"fdd70777-e9cf-4317-afb6-cae87f75d5b0\"},{\"content\":{\"connectorIds\":[\"RConn1\"],\"side\":\"BOTTOM\"},\"type\":\"ConnectorPlacement.EquallySpacedRectSide\",\"uuid\":\"2353ed68-b1a1-4775-9ca9-31e268d5443b\"}]},\"type\":\"ConnectorPlacement.EquallySpacedConnector\",\"uuid\":\"d5479f4c-4e65-4791-adcb-73df11f88590\"}],\"packageUris\":[\"http://schema.mathworks.com/mf0/Connector/R2020b\"],\"version\":\"1.0\"}"
  Udc(+) : PMIOPort  Side=Left
  us_u : PMIOPort  Port=2  Side=Right
  Udc(-) : PMIOPort  Port=3  Side=Left
  wires:
  [inv_mu_top] -> Simulink-PS Converter/1
  [inv_mu_bottom] -> Simulink-PS Converter1/1
  connections:
  Udc(+)/RConn1 -- switch_1/LConn2
  switch_2/LConn1 -- Simulink-PS Converter1/RConn1
  Simulink-PS Converter/RConn1 -- switch_1/LConn1
  us_u/RConn1 -- switch_2/LConn2 -- switch_1/RConn1
  Udc(-)/RConn1 -- switch_2/RConn1

== system afe_rst_inv_psm_distributed_control_two_delays/INV-Modular/inv_leg_v/dclink_measure ==
  Controlled Voltage Source : fl_lib/Electrical/Electrical Sources/Controlled Voltage Source
  Current Sensor1 : fl_lib/Electrical/Electrical Sensors/Current Sensor
  Electrical Reference : fl_lib/Electrical/Electrical Elements/Electrical Reference
  Gain : Gain  Gain=107.5e3
  Gain1 : Gain  Gain=1/Vdc_bez
  Quantizer : Quantizer  QuantizationInterval=VoltageQuantization
  Resistor : fl_lib/Electrical/Electrical Elements/Resistor  R=107.5 kOhm  i_specify=off  i_priority=None  i=0 A  i_nominal_specify=off  i_nominal_value=1  i_nominal_unit=A  v_specify=off  v_priority=None  v=0 V  v_nominal_specify=off  v_nominal_value=1  v_nominal_unit=V
  Saturation : Saturate  UpperLimit=inf  LowerLimit=1
  im_udc : nesl_utility/PS-Simulink Converter  PhysicalDomain=network_engine_domain  SubClassName=ps_output  LeftPortType=input  RightPortType=output  PseudoPeriodic=off  Frequencies=[]  VectorFormat=1-D array  Unit=A  AffineConversion=on
  udc : PMIOPort  Side=Left
  tag scope: udc_dbv=global, udc_pu_dbv=global
  wires:
  Gain/1 -> [udc_dbv], Saturation/1
  Quantizer/1 -> Gain1/1
  Saturation/1 -> Quantizer/1
  im_udc/1 -> Gain/1
  Gain1/1 -> [udc_pu_dbv]
  connections:
  udc/RConn1 -- Controlled Voltage Source/RConn1
  Current Sensor1/RConn1 -- im_udc/LConn1
  Current Sensor1/RConn2 -- Electrical Reference/LConn1 -- Controlled Voltage Source/RConn2
  Resistor/RConn1 -- Current Sensor1/LConn1
  Controlled Voltage Source/LConn1 -- Resistor/LConn1

== system afe_rst_inv_psm_distributed_control_two_delays/INV-Modular/inv_leg_v/driver_board_v ==
  double_integrator_observer : Subsystem
  motor_vector_control : Subsystem
  voltage-current-acquisition : Subsystem
  us_alphabeta_ctrl : Outport
  tag scope: motor_phase_mb_fb_dbv_luenberger=global
  wires:
  motor_vector_control/1(us_alphabeta_ctrl) -> us_alphabeta_ctrl/1
  [motor_torque_ref_dbu_fb_dbv] -> motor_vector_control/1(motor_torque_ref)
  [motor_phase_mb_fb_dbv] -> double_integrator_observer/1(theta)
  double_integrator_observer/2(theta_hat) -> [motor_phase_mb_fb_dbv_luenberger]  "theta_hat"

== system afe_rst_inv_psm_distributed_control_two_delays/INV-Modular/inv_leg_v/modulator ==
  us_alphabeta_ctrl : Inport
  Bus Selector : BusSelector  OutputSignals=pwm_v_top,pwm_v_bottom
  Constant1 : Constant
  sv_pwm : Subsystem
  tag scope: inv_mv_bottom=global, inv_mv_top=global
  wires:
  Bus Selector/2 -> [inv_mv_bottom]  "<pwm_v_bottom>"
  us_alphabeta_ctrl/1 -> sv_pwm/1(ab)
  Bus Selector/1 -> [inv_mv_top]  "<pwm_v_top>"
  Constant1/1 -> sv_pwm/2(enable)
  sv_pwm/1(firing_gates) -> Bus Selector/1

== system afe_rst_inv_psm_distributed_control_two_delays/INV-Modular/inv_leg_v/solid_state_inverter ==
  Simulink-PS Converter : nesl_utility/Simulink-PS Converter  PhysicalDomain=network_engine_domain  SubClassName=ps_input  LeftPortType=input  RightPortType=output  PseudoPeriodic=off  Frequencies=[]  NoiseDistribution=none  NoiseParameters=[]  Unit=1  AffineConversion=off  FilteringAndDerivatives=provide  SimscapeFilterOrder=1  InputFilterTimeConstant=0.001  UdotUserProvided=0
  Simulink-PS Converter1 : nesl_utility/Simulink-PS Converter  PhysicalDomain=network_engine_domain  SubClassName=ps_input  LeftPortType=input  RightPortType=output  PseudoPeriodic=off  Frequencies=[]  NoiseDistribution=none  NoiseParameters=[]  Unit=1  AffineConversion=off  FilteringAndDerivatives=provide  SimscapeFilterOrder=1  InputFilterTimeConstant=0.001  UdotUserProvided=0
  switch_1 : Subsystem
      settings: PortSchema="{\"entries\":[{\"content\":{\"sides\":[{\"content\":{\"connectorIds\":[\"LConn1\"]},\"type\":\"ConnectorPlacement.EquallySpacedRectSide\",\"uuid\":\"9277da8d-d460-43e6-8478-dd662f15d226\"},{\"content\":{\"connectorIds\":[],\"side\":\"RIGHT\"},\"type\":\"ConnectorPlacement.EquallySpacedRectSide\",\"uuid\":\"a7ece396-f1d9-4f4f-a05b-db1fc65d6e1d\"},{\"content\":{\"connectorIds\":[\"LConn2\"],\"side\":\"TOP\"},\"type\":\"ConnectorPlacement.EquallySpacedRectSide\",\"uuid\":\"fdd70777-e9cf-4317-afb6-cae87f75d5b0\"},{\"content\":{\"connectorIds\":[\"RConn1\"],\"side\":\"BOTTOM\"},\"type\":\"ConnectorPlacement.EquallySpacedRectSide\",\"uuid\":\"2353ed68-b1a1-4775-9ca9-31e268d5443b\"}]},\"type\":\"ConnectorPlacement.EquallySpacedConnector\",\"uuid\":\"d5479f4c-4e65-4791-adcb-73df11f88590\"}],\"packageUris\":[\"http://schema.mathworks.com/mf0/Connector/R2020b\"],\"version\":\"1.0\"}"
  switch_2 : Subsystem
      settings: PortSchema="{\"entries\":[{\"content\":{\"sides\":[{\"content\":{\"connectorIds\":[\"LConn1\"]},\"type\":\"ConnectorPlacement.EquallySpacedRectSide\",\"uuid\":\"9277da8d-d460-43e6-8478-dd662f15d226\"},{\"content\":{\"connectorIds\":[],\"side\":\"RIGHT\"},\"type\":\"ConnectorPlacement.EquallySpacedRectSide\",\"uuid\":\"a7ece396-f1d9-4f4f-a05b-db1fc65d6e1d\"},{\"content\":{\"connectorIds\":[\"LConn2\"],\"side\":\"TOP\"},\"type\":\"ConnectorPlacement.EquallySpacedRectSide\",\"uuid\":\"fdd70777-e9cf-4317-afb6-cae87f75d5b0\"},{\"content\":{\"connectorIds\":[\"RConn1\"],\"side\":\"BOTTOM\"},\"type\":\"ConnectorPlacement.EquallySpacedRectSide\",\"uuid\":\"2353ed68-b1a1-4775-9ca9-31e268d5443b\"}]},\"type\":\"ConnectorPlacement.EquallySpacedConnector\",\"uuid\":\"d5479f4c-4e65-4791-adcb-73df11f88590\"}],\"packageUris\":[\"http://schema.mathworks.com/mf0/Connector/R2020b\"],\"version\":\"1.0\"}"
  Udc(+) : PMIOPort  Side=Left
  us_u : PMIOPort  Port=2  Side=Right
  Udc(-) : PMIOPort  Port=3  Side=Left
  wires:
  [inv_mv_bottom] -> Simulink-PS Converter1/1
  [inv_mv_top] -> Simulink-PS Converter/1
  connections:
  Udc(-)/RConn1 -- switch_2/RConn1
  switch_1/RConn1 -- switch_2/LConn2 -- us_u/RConn1
  Simulink-PS Converter/RConn1 -- switch_1/LConn1
  switch_2/LConn1 -- Simulink-PS Converter1/RConn1
  Udc(+)/RConn1 -- switch_1/LConn2

== system afe_rst_inv_psm_distributed_control_two_delays/INV-Modular/inv_leg_w/dclink_measure ==
  Controlled Voltage Source : fl_lib/Electrical/Electrical Sources/Controlled Voltage Source
  Current Sensor1 : fl_lib/Electrical/Electrical Sensors/Current Sensor
  Electrical Reference : fl_lib/Electrical/Electrical Elements/Electrical Reference
  Gain : Gain  Gain=107.5e3
  Gain1 : Gain  Gain=1/Vdc_bez
  Quantizer : Quantizer  QuantizationInterval=VoltageQuantization
  Resistor : fl_lib/Electrical/Electrical Elements/Resistor  R=107.5 kOhm  i_specify=off  i_priority=None  i=0 A  i_nominal_specify=off  i_nominal_value=1  i_nominal_unit=A  v_specify=off  v_priority=None  v=0 V  v_nominal_specify=off  v_nominal_value=1  v_nominal_unit=V
  Saturation : Saturate  UpperLimit=inf  LowerLimit=1
  im_udc : nesl_utility/PS-Simulink Converter  PhysicalDomain=network_engine_domain  SubClassName=ps_output  LeftPortType=input  RightPortType=output  PseudoPeriodic=off  Frequencies=[]  VectorFormat=1-D array  Unit=A  AffineConversion=on
  udc : PMIOPort  Side=Left
  tag scope: udc_pu_dbw=global
  wires:
  Gain/1 -> Saturation/1
  Quantizer/1 -> Gain1/1
  Saturation/1 -> Quantizer/1
  im_udc/1 -> Gain/1
  Gain1/1 -> [udc_pu_dbw]
  connections:
  udc/RConn1 -- Controlled Voltage Source/RConn1
  Current Sensor1/RConn1 -- im_udc/LConn1
  Current Sensor1/RConn2 -- Electrical Reference/LConn1 -- Controlled Voltage Source/RConn2
  Resistor/RConn1 -- Current Sensor1/LConn1
  Controlled Voltage Source/LConn1 -- Resistor/LConn1

== system afe_rst_inv_psm_distributed_control_two_delays/INV-Modular/inv_leg_w/driver_board_w ==
  double_integrator_observer : Subsystem
  motor_vector_control : Subsystem
  voltage-current-acquisition : Subsystem
  us_alphabeta_ctrl : Outport
  tag scope: motor_phase_mb_fb_dbw_luenberger=global
  wires:
  [motor_torque_ref_dbu_fb_dbw] -> motor_vector_control/1(motor_torque_ref)
  motor_vector_control/1(us_alphabeta_ctrl) -> us_alphabeta_ctrl/1
  [motor_phase_mb_fb_dbw] -> double_integrator_observer/1(theta)
  double_integrator_observer/2(theta_hat) -> [motor_phase_mb_fb_dbw_luenberger]  "theta_hat"

== system afe_rst_inv_psm_distributed_control_two_delays/INV-Modular/inv_leg_w/modulator ==
  u_alphabeta_ctrl : Inport
  Bus Selector : BusSelector  OutputSignals=pwm_w_top,pwm_w_bottom
  Constant1 : Constant
  sv_pwm : Subsystem
  tag scope: inv_mw_bottom=global, inv_mw_top=global
  wires:
  sv_pwm/1(firing_gates) -> Bus Selector/1
  Constant1/1 -> sv_pwm/2(enable)
  Bus Selector/1 -> [inv_mw_top]  "<pwm_w_top>"
  u_alphabeta_ctrl/1 -> sv_pwm/1(u_alphabeta_ctrl)
  Bus Selector/2 -> [inv_mw_bottom]  "<pwm_w_bottom>"

== system afe_rst_inv_psm_distributed_control_two_delays/INV-Modular/inv_leg_w/solid_state_inverter ==
  Simulink-PS Converter : nesl_utility/Simulink-PS Converter  PhysicalDomain=network_engine_domain  SubClassName=ps_input  LeftPortType=input  RightPortType=output  PseudoPeriodic=off  Frequencies=[]  NoiseDistribution=none  NoiseParameters=[]  Unit=1  AffineConversion=off  FilteringAndDerivatives=provide  SimscapeFilterOrder=1  InputFilterTimeConstant=0.001  UdotUserProvided=0
  Simulink-PS Converter1 : nesl_utility/Simulink-PS Converter  PhysicalDomain=network_engine_domain  SubClassName=ps_input  LeftPortType=input  RightPortType=output  PseudoPeriodic=off  Frequencies=[]  NoiseDistribution=none  NoiseParameters=[]  Unit=1  AffineConversion=off  FilteringAndDerivatives=provide  SimscapeFilterOrder=1  InputFilterTimeConstant=0.001  UdotUserProvided=0
  switch_1 : Subsystem
      settings: PortSchema="{\"entries\":[{\"content\":{\"sides\":[{\"content\":{\"connectorIds\":[\"LConn1\"]},\"type\":\"ConnectorPlacement.EquallySpacedRectSide\",\"uuid\":\"9277da8d-d460-43e6-8478-dd662f15d226\"},{\"content\":{\"connectorIds\":[],\"side\":\"RIGHT\"},\"type\":\"ConnectorPlacement.EquallySpacedRectSide\",\"uuid\":\"a7ece396-f1d9-4f4f-a05b-db1fc65d6e1d\"},{\"content\":{\"connectorIds\":[\"LConn2\"],\"side\":\"TOP\"},\"type\":\"ConnectorPlacement.EquallySpacedRectSide\",\"uuid\":\"fdd70777-e9cf-4317-afb6-cae87f75d5b0\"},{\"content\":{\"connectorIds\":[\"RConn1\"],\"side\":\"BOTTOM\"},\"type\":\"ConnectorPlacement.EquallySpacedRectSide\",\"uuid\":\"2353ed68-b1a1-4775-9ca9-31e268d5443b\"}]},\"type\":\"ConnectorPlacement.EquallySpacedConnector\",\"uuid\":\"d5479f4c-4e65-4791-adcb-73df11f88590\"}],\"packageUris\":[\"http://schema.mathworks.com/mf0/Connector/R2020b\"],\"version\":\"1.0\"}"
  switch_2 : Subsystem
      settings: PortSchema="{\"entries\":[{\"content\":{\"sides\":[{\"content\":{\"connectorIds\":[\"LConn1\"]},\"type\":\"ConnectorPlacement.EquallySpacedRectSide\",\"uuid\":\"9277da8d-d460-43e6-8478-dd662f15d226\"},{\"content\":{\"connectorIds\":[],\"side\":\"RIGHT\"},\"type\":\"ConnectorPlacement.EquallySpacedRectSide\",\"uuid\":\"a7ece396-f1d9-4f4f-a05b-db1fc65d6e1d\"},{\"content\":{\"connectorIds\":[\"LConn2\"],\"side\":\"TOP\"},\"type\":\"ConnectorPlacement.EquallySpacedRectSide\",\"uuid\":\"fdd70777-e9cf-4317-afb6-cae87f75d5b0\"},{\"content\":{\"connectorIds\":[\"RConn1\"],\"side\":\"BOTTOM\"},\"type\":\"ConnectorPlacement.EquallySpacedRectSide\",\"uuid\":\"2353ed68-b1a1-4775-9ca9-31e268d5443b\"}]},\"type\":\"ConnectorPlacement.EquallySpacedConnector\",\"uuid\":\"d5479f4c-4e65-4791-adcb-73df11f88590\"}],\"packageUris\":[\"http://schema.mathworks.com/mf0/Connector/R2020b\"],\"version\":\"1.0\"}"
  Udc(+) : PMIOPort  Side=Left
  us_b : PMIOPort  Port=2  Side=Right
  Udc(-) : PMIOPort  Port=3  Side=Left
  wires:
  [inv_mw_top] -> Simulink-PS Converter/1
  [inv_mw_bottom] -> Simulink-PS Converter1/1
  connections:
  Udc(+)/RConn1 -- switch_1/LConn2
  switch_2/LConn1 -- Simulink-PS Converter1/RConn1
  Simulink-PS Converter/RConn1 -- switch_1/LConn1
  switch_2/LConn2 -- us_b/RConn1 -- switch_1/RConn1
  Udc(-)/RConn1 -- switch_2/RConn1

== system afe_rst_inv_psm_distributed_control_two_delays/grid/grid_emulator/3ph_YYg ==
  Electrical Reference1 : fl_lib/Electrical/Electrical Elements/Electrical Reference
  ph1 : single_phase_transformer_lib/single phase transformer  Lm=Lmu2_trafo H  n1=1  n2=1  Rd1=0 Ohm  Rd2=Rd2_trafo Ohm  Ld1=0 H  Ld2=Ld2_trafo H  Rfe=Rm2_trafo Ohm  phi_specify=off  phi_priority=None  phi=0 V*s  phi_nominal_specify=off  phi_nominal_value=1  phi_nominal_unit=V*s  i1_specify=off  i1_priority=None  i1=0 A  i1_nominal_specify=off  i1_nominal_value=1  i1_nominal_unit=A  i2_specify=off  i2_priority=None  i2=0 A  i2_nominal_specify=off  i2_nominal_value=1  i2_nominal_unit=A  ife_specify=off  ife_priority=None  ife=0 A  ife_nominal_specify=off  ife_nominal_value=1  ife_nominal_unit=A  u1_specify=off  u1_priority=None  u1=0 V  u1_nominal_specify=off  u1_nominal_value=1  u1_nominal_unit=V  u2_specify=off  u2_priority=None  u2=0 V  u2_nominal_specify=off  u2_nominal_value=1  u2_nominal_unit=V
  ph2 : single_phase_transformer_lib/single phase transformer  Lm=Lmu2_trafo H  n1=1  n2=1  Rd1=0 Ohm  Rd2=Rd2_trafo Ohm  Ld1=0 H  Ld2=Ld2_trafo H  Rfe=Rm2_trafo Ohm  phi_specify=off  phi_priority=None  phi=0 V*s  phi_nominal_specify=off  phi_nominal_value=1  phi_nominal_unit=V*s  i1_specify=off  i1_priority=None  i1=0 A  i1_nominal_specify=off  i1_nominal_value=1  i1_nominal_unit=A  i2_specify=off  i2_priority=None  i2=0 A  i2_nominal_specify=off  i2_nominal_value=1  i2_nominal_unit=A  ife_specify=off  ife_priority=None  ife=0 A  ife_nominal_specify=off  ife_nominal_value=1  ife_nominal_unit=A  u1_specify=off  u1_priority=None  u1=0 V  u1_nominal_specify=off  u1_nominal_value=1  u1_nominal_unit=V  u2_specify=off  u2_priority=None  u2=0 V  u2_nominal_specify=off  u2_nominal_value=1  u2_nominal_unit=V
  ph3 : single_phase_transformer_lib/single phase transformer  Lm=Lmu2_trafo H  n1=1  n2=1  Rd1=0 Ohm  Rd2=Rd2_trafo Ohm  Ld1=0 H  Ld2=Ld2_trafo H  Rfe=Rm2_trafo Ohm  phi_specify=off  phi_priority=None  phi=0 V*s  phi_nominal_specify=off  phi_nominal_value=1  phi_nominal_unit=V*s  i1_specify=off  i1_priority=None  i1=0 A  i1_nominal_specify=off  i1_nominal_value=1  i1_nominal_unit=A  i2_specify=off  i2_priority=None  i2=0 A  i2_nominal_specify=off  i2_nominal_value=1  i2_nominal_unit=A  ife_specify=off  ife_priority=None  ife=0 A  ife_nominal_specify=off  ife_nominal_value=1  ife_nominal_unit=A  u1_specify=off  u1_priority=None  u1=0 V  u1_nominal_specify=off  u1_nominal_value=1  u1_nominal_unit=V  u2_specify=off  u2_priority=None  u2=0 V  u2_nominal_specify=off  u2_nominal_value=1  u2_nominal_unit=V
  ua : PMIOPort  Side=Right
  ub : PMIOPort  Port=2  Side=Right
  uc : PMIOPort  Port=3  Side=Right
  Ua : PMIOPort  Port=4  Side=Left
  Ub : PMIOPort  Port=5  Side=Left
  Uc : PMIOPort  Port=6  Side=Left
  connections:
  Electrical Reference1/LConn1 -- ph3/RConn2 -- ph2/RConn2 -- ph1/RConn2
  uc/RConn1 -- ph3/RConn1
  ph1/LConn1 -- Ua/RConn1
  ph3/LConn1 -- Uc/RConn1
  ph1/RConn1 -- ua/RConn1
  ph2/RConn1 -- ub/RConn1
  ph2/LConn1 -- Ub/RConn1
  ph1/LConn2 -- ph3/LConn2 -- ph2/LConn2

== system afe_rst_inv_psm_distributed_control_two_delays/grid/grid_emulator/grid_emulator ==
  phase_gen : Subsystem
  voltage_reference : Subsystem
  voltage_source : Subsystem
  Vma : Outport
  Vmb : Outport  Port=2
  Vmc : Outport  Port=3
  wires:
  phase_gen/1(grid_emu_phase) -> voltage_reference/1(grid_emu_phase)  "grid_emu_phase"
  voltage_source/2(vn_xi) -> voltage_reference/3(Vxi_n)
  voltage_source/1(vp_xi) -> voltage_reference/2(Vxi_p)
  voltage_source/3(vn_eta) -> voltage_reference/4(Veta_n)
  voltage_reference/1(V1_ref1) -> Vma/1
  voltage_reference/2(V2_ref1) -> Vmb/1
  voltage_reference/3(V3_ref1) -> Vmc/1

== system afe_rst_inv_psm_distributed_control_two_delays/grid/grid_emulator/threephase_vi_measures ==
  Bus Creator : BusCreator  Inputs=6
  Current Sensor : fl_lib/Electrical/Electrical Sensors/Current Sensor
  Current Sensor1 : fl_lib/Electrical/Electrical Sensors/Current Sensor
  Current Sensor2 : fl_lib/Electrical/Electrical Sensors/Current Sensor
  Electrical Reference1 : fl_lib/Electrical/Electrical Elements/Electrical Reference
  Voltage Sensor : fl_lib/Electrical/Electrical Sensors/Voltage Sensor
  Voltage Sensor1 : fl_lib/Electrical/Electrical Sensors/Voltage Sensor
  Voltage Sensor2 : fl_lib/Electrical/Electrical Sensors/Voltage Sensor
  i : Selector  InputPortWidth=6  IndexOptions=Index vector (dialog)  Indices=[4 5 6]  OutputSizes=1
  i_line_abc/u_line_abc : Scope  NumInputPorts=2
      settings: SampleTime=tc  ActiveDisplayYMinimum=-6158.56909  ActiveDisplayYMaximum=6444.00805  DataLoggingVariableName=ScopeData2
  ia_grid : nesl_utility/PS-Simulink Converter  PhysicalDomain=network_engine_domain  SubClassName=ps_output  LeftPortType=input  RightPortType=output  PseudoPeriodic=off  Frequencies=[]  VectorFormat=1-D array  Unit=A  AffineConversion=off
  ib_grid : nesl_utility/PS-Simulink Converter  PhysicalDomain=network_engine_domain  SubClassName=ps_output  LeftPortType=input  RightPortType=output  PseudoPeriodic=off  Frequencies=[]  VectorFormat=1-D array  Unit=A  AffineConversion=off
  ic_grid : nesl_utility/PS-Simulink Converter  PhysicalDomain=network_engine_domain  SubClassName=ps_output  LeftPortType=input  RightPortType=output  PseudoPeriodic=off  Frequencies=[]  VectorFormat=1-D array  Unit=A  AffineConversion=off
  u : Selector  InputPortWidth=6  IndexOptions=Index vector (dialog)  Indices=[1 2 3]  OutputSizes=1
  ua_grid : nesl_utility/PS-Simulink Converter  PhysicalDomain=network_engine_domain  SubClassName=ps_output  LeftPortType=input  RightPortType=output  PseudoPeriodic=off  Frequencies=[]  VectorFormat=1-D array  Unit=V  AffineConversion=off
  ub_grid : nesl_utility/PS-Simulink Converter  PhysicalDomain=network_engine_domain  SubClassName=ps_output  LeftPortType=input  RightPortType=output  PseudoPeriodic=off  Frequencies=[]  VectorFormat=1-D array  Unit=V  AffineConversion=off
  uc_grid : nesl_utility/PS-Simulink Converter  PhysicalDomain=network_engine_domain  SubClassName=ps_output  LeftPortType=input  RightPortType=output  PseudoPeriodic=off  Frequencies=[]  VectorFormat=1-D array  Unit=V  AffineConversion=off
  Ua : PMIOPort  Side=Left
  ua : PMIOPort  Port=2  Side=Right
  Ub : PMIOPort  Port=3  Side=Left
  ub : PMIOPort  Port=4  Side=Right
  Uc : PMIOPort  Port=5  Side=Left
  uc : PMIOPort  Port=6  Side=Right
  wires:
  Bus Creator/1 -> i/1, u/1  "vi_data"
  ib_grid/1 -> Bus Creator/5  "ib"
  ia_grid/1 -> Bus Creator/4  "ia"
  ic_grid/1 -> Bus Creator/6  "ic"
  ua_grid/1 -> Bus Creator/1  "ua"
  ub_grid/1 -> Bus Creator/2  "ub"
  uc_grid/1 -> Bus Creator/3  "uc"
  i/1 -> i_line_abc/u_line_abc/1
  u/1 -> i_line_abc/u_line_abc/2
  connections:
  Current Sensor1/LConn1 -- Ub/RConn1 -- Voltage Sensor1/LConn1
  Electrical Reference1/LConn1 -- Voltage Sensor/RConn2 -- Voltage Sensor2/RConn2 -- Voltage Sensor1/RConn2
  Voltage Sensor/RConn1 -- ua_grid/LConn1
  Current Sensor/RConn2 -- ua/RConn1
  Voltage Sensor1/RConn1 -- ub_grid/LConn1
  Voltage Sensor2/LConn1 -- Current Sensor2/LConn1 -- Uc/RConn1
  Current Sensor/LConn1 -- Ua/RConn1 -- Voltage Sensor/LConn1
  Current Sensor1/RConn2 -- ub/RConn1
  Voltage Sensor2/RConn1 -- uc_grid/LConn1
  ib_grid/LConn1 -- Current Sensor1/RConn1
  ia_grid/LConn1 -- Current Sensor/RConn1
  ic_grid/LConn1 -- Current Sensor2/RConn1
  Current Sensor2/RConn2 -- uc/RConn1

== system afe_rst_inv_psm_distributed_control_two_delays/grid/instantaneus_power/abc2alphabeta ==
  a : Inport
  b : Inport  Port=2
  c : Inport  Port=3
  abc2alphabeta : Subsystem
  vline_alpha : Outport  VectorParamsAs1DForOutWhenUnconnected=off
  vline_beta : Outport  Port=2  VectorParamsAs1DForOutWhenUnconnected=off
  wires:
  a/1 -> abc2alphabeta/1(a)
  b/1 -> abc2alphabeta/2(b)
  c/1 -> abc2alphabeta/3(c)
  abc2alphabeta/2("beta ") -> vline_beta/1
  abc2alphabeta/1("alpha ") -> vline_alpha/1

== system afe_rst_inv_psm_distributed_control_two_delays/grid/instantaneus_power/abc2alphabeta  ==
  a : Inport
  b : Inport  Port=2
  c : Inport  Port=3
  abc->alphabeta : Subsystem
  i_line_alpha : Outport  VectorParamsAs1DForOutWhenUnconnected=off
  i_line_beta : Outport  Port=2  VectorParamsAs1DForOutWhenUnconnected=off
  wires:
  abc->alphabeta/1("alpha ") -> i_line_alpha/1
  abc->alphabeta/2("beta ") -> i_line_beta/1
  c/1 -> abc->alphabeta/3(c)
  b/1 -> abc->alphabeta/2(b)
  a/1 -> abc->alphabeta/1(a)

== system afe_rst_inv_psm_distributed_control_two_delays/grid/instantaneus_power/moving_avarage ==
  In : Inport
  Gain1 : Gain  Gain=omega_grid_emulator_nom/2/pi  SaturateOnIntegerOverflow=on  OutDataTypeStr=Inherit: Same as input  ParamDataTypeStr=Inherit: Same as input
  Sum4 : Sum  SaturateOnIntegerOverflow=on
  Sum8 : Sum  Inputs=+-  InputSameDT=on  SaturateOnIntegerOverflow=on  OutDataTypeStr=Inherit: Same as first input
  Transport Delay : TransportDelay  DelayTime=2*pi/omega_grid_emulator_nom  BufferSize=2048*4  PadeOrder=2
  Unit Delay2 : UnitDelay  SampleTime=ts_afe
  kp2 : Gain  Gain=ts_afe  SaturateOnIntegerOverflow=on  OutDataTypeStr=Inherit: Same as input  ParamDataTypeStr=Inherit: Same as input
  Mean : Outport  VectorParamsAs1DForOutWhenUnconnected=off
  wires:
  Transport Delay/1 -> Sum8/2
  Sum4/1 -> Sum8/1, Transport Delay/1, Unit Delay2/1
  Sum8/1 -> Gain1/1
  In/1 -> kp2/1
  Unit Delay2/1 -> Sum4/2
  kp2/1 -> Sum4/1
  Gain1/1 -> Mean/1
